simulink model "dcdc_zvs_full_bridge"  (R2026b)
settings: Solver=ode23tb  StopTime=simlength  FixedStep=tc  MaxStep=tc
values from neighbouring files (symbols this model uses):
  Idc_FS = max(Idab1_dc_nom,Idab2_dc_nom) * margin_factor    [init_model.m]
  L_core_length = 95    [magnetics_design_transformer.m]
  number_of_cells_2_sim = floor((Uout_nom-delta_load)/u_cell)    [init_model.m]    (also in run_sim_output_current_ctrl.m = floor((Uout_max-delta_load)/u_cell))
  Pnom = 175e3    (= 175000)    [init_model.m]
  tc = ts_dab/400    (= 5e-07)    [init_model.m]
  u_cell = 3.6    [init_model.m]
  Vdab2_dc_nom = ubattery2    (= 540)    [init_model.m]
  Vdc_FS = max(Vdab1_dc_nom,Vdab2_dc_nom) * margin_factor    [init_model.m]
libraries: fl_lib x32, nesl_utility x22, discrete_time_low_pass_filter x7, lithium_ion_battery x2, pi_ctrl x2, full_bridge_diode_rectifier x2, full_bridge_zvs_pwm_modulator x1, full_bridge_ideal_switch x1, full_bridge_igbt_based_with_thermal_model x1, full_bridge_mosfet_based_with_thermal_model_zvs x1, three_windings_transformer x1
(part 2 of 2)

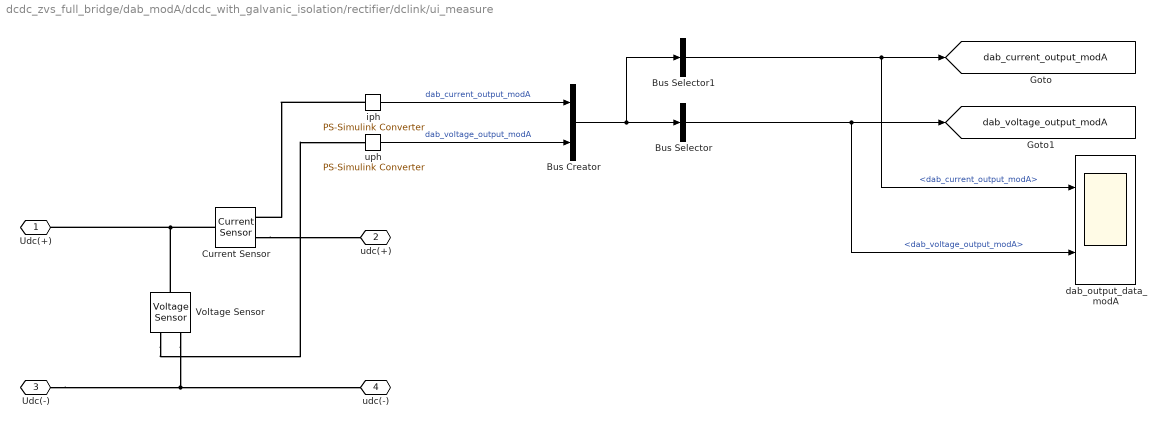
== system dcdc_zvs_full_bridge/dab_modA/dcdc_with_galvanic_isolation/rectifier/dclink/ui_measure ==
  Bus Creator : BusCreator  Inputs=2
  Bus Selector : BusSelector  OutputSignals=dab_voltage_output_modA
  Bus Selector1 : BusSelector  OutputSignals=dab_current_output_modA
  Current Sensor : fl_lib/Electrical/Electrical Sensors/Current Sensor
  Voltage Sensor : fl_lib/Electrical/Electrical Sensors/Voltage Sensor
  dab_output_data_modA : Scope  NumInputPorts=2
      settings: SampleTime=tc  ActiveDisplayYMinimum=283.61167297568261  ActiveDisplayYMaximum=358.14263055151184  DataLoggingVariableName=ScopeData11
  iph : nesl_utility/PS-Simulink Converter  PhysicalDomain=network_engine_domain  SubClassName=ps_output  LeftPortType=input  RightPortType=output  PseudoPeriodic=off  Frequencies=[]  VectorFormat=1-D array  Unit=A  AffineConversion=off
  uph : nesl_utility/PS-Simulink Converter  PhysicalDomain=network_engine_domain  SubClassName=ps_output  LeftPortType=input  RightPortType=output  PseudoPeriodic=off  Frequencies=[]  VectorFormat=1-D array  Unit=V  AffineConversion=off
  Udc(+) : PMIOPort  Side=Left
  udc(+) : PMIOPort  Port=2  Side=Right
  Udc(-) : PMIOPort  Port=3  Side=Left
  udc(-) : PMIOPort  Port=4  Side=Right
  tag scope: dab_current_output_modA=global, dab_voltage_output_modA=global
  wires:
  Bus Creator/1 -> Bus Selector1/1, Bus Selector/1
  iph/1 -> Bus Creator/1  "dab_current_output_modA"
  uph/1 -> Bus Creator/2  "dab_voltage_output_modA"
  Bus Selector1/1 -> [dab_current_output_modA], dab_output_data_modA/1  "<dab_current_output_modA>"
  Bus Selector/1 -> [dab_voltage_output_modA], dab_output_data_modA/2  "<dab_voltage_output_modA>"
  connections:
  iph/LConn1 -- Current Sensor/RConn1
  Voltage Sensor/LConn1 -- Current Sensor/LConn1 -- Udc(+)/RConn1
  Current Sensor/RConn2 -- udc(+)/RConn1
  Voltage Sensor/RConn1 -- uph/LConn1
  Voltage Sensor/RConn2 -- Udc(-)/RConn1 -- udc(-)/RConn1

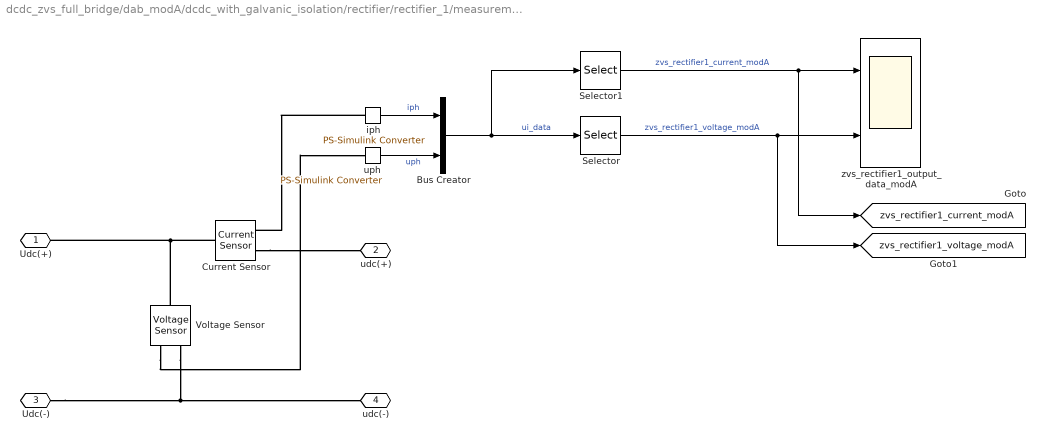
== system dcdc_zvs_full_bridge/dab_modA/dcdc_with_galvanic_isolation/rectifier/rectifier_1/measurements_rectifier_output_1 ==
  Bus Creator : BusCreator  Inputs=2
  Current Sensor : fl_lib/Electrical/Electrical Sensors/Current Sensor
  Selector : Selector  InputPortWidth=2  IndexOptions=Index vector (dialog)  Indices=2  OutputSizes=1  RuntimeRangeChecks=off
  Selector1 : Selector  InputPortWidth=2  IndexOptions=Index vector (dialog)  Indices=1  OutputSizes=1  RuntimeRangeChecks=off
  Voltage Sensor : fl_lib/Electrical/Electrical Sensors/Voltage Sensor
  iph : nesl_utility/PS-Simulink Converter  PhysicalDomain=network_engine_domain  SubClassName=ps_output  LeftPortType=input  RightPortType=output  PseudoPeriodic=off  Frequencies=[]  VectorFormat=1-D array  Unit=A  AffineConversion=off
  uph : nesl_utility/PS-Simulink Converter  PhysicalDomain=network_engine_domain  SubClassName=ps_output  LeftPortType=input  RightPortType=output  PseudoPeriodic=off  Frequencies=[]  VectorFormat=1-D array  Unit=V  AffineConversion=off
  zvs_rectifier1_output_data_modA : Scope  NumInputPorts=2
      settings: SampleTime=tc  ActiveDisplayYMinimum=-126.83833202722374  ActiveDisplayYMaximum=1141.4829766347427  DataLoggingVariableName=ScopeData2
  Udc(+) : PMIOPort  Side=Left
  udc(+) : PMIOPort  Port=2  Side=Right
  Udc(-) : PMIOPort  Port=3  Side=Left
  udc(-) : PMIOPort  Port=4  Side=Right
  tag scope: zvs_rectifier1_current_modA=global, zvs_rectifier1_voltage_modA=global
  wires:
  Bus Creator/1 -> Selector/1, Selector1/1  "ui_data"
  iph/1 -> Bus Creator/1  "iph"
  uph/1 -> Bus Creator/2  "uph"
  Selector1/1 -> [zvs_rectifier1_current_modA], zvs_rectifier1_output_data_modA/1  "zvs_rectifier1_current_modA"
  Selector/1 -> [zvs_rectifier1_voltage_modA], zvs_rectifier1_output_data_modA/2  "zvs_rectifier1_voltage_modA"
  connections:
  iph/LConn1 -- Current Sensor/RConn1
  Voltage Sensor/LConn1 -- Current Sensor/LConn1 -- Udc(+)/RConn1
  Current Sensor/RConn2 -- udc(+)/RConn1
  Voltage Sensor/RConn1 -- uph/LConn1
  Voltage Sensor/RConn2 -- Udc(-)/RConn1 -- udc(-)/RConn1

== system dcdc_zvs_full_bridge/dab_modA/dcdc_with_galvanic_isolation/rectifier/rectifier_2/measurements_rectifier_output_1 ==
  Bus Creator : BusCreator  Inputs=2
  Current Sensor : fl_lib/Electrical/Electrical Sensors/Current Sensor
  Selector : Selector  InputPortWidth=2  IndexOptions=Index vector (dialog)  Indices=2  OutputSizes=1  RuntimeRangeChecks=off
  Selector1 : Selector  InputPortWidth=2  IndexOptions=Index vector (dialog)  Indices=1  OutputSizes=1  RuntimeRangeChecks=off
  Voltage Sensor : fl_lib/Electrical/Electrical Sensors/Voltage Sensor
  iph : nesl_utility/PS-Simulink Converter  PhysicalDomain=network_engine_domain  SubClassName=ps_output  LeftPortType=input  RightPortType=output  PseudoPeriodic=off  Frequencies=[]  VectorFormat=1-D array  Unit=A  AffineConversion=off
  uph : nesl_utility/PS-Simulink Converter  PhysicalDomain=network_engine_domain  SubClassName=ps_output  LeftPortType=input  RightPortType=output  PseudoPeriodic=off  Frequencies=[]  VectorFormat=1-D array  Unit=V  AffineConversion=off
  zvs_rectifier1_output_data_modA : Scope  NumInputPorts=2
      settings: SampleTime=tc  ActiveDisplayYMinimum=-126.83833202722374  ActiveDisplayYMaximum=1141.4829766347427  DataLoggingVariableName=ScopeData2
  Udc(+) : PMIOPort  Side=Left
  udc(+) : PMIOPort  Port=2  Side=Right
  Udc(-) : PMIOPort  Port=3  Side=Left
  udc(-) : PMIOPort  Port=4  Side=Right
  tag scope: zvs_rectifier2_current_modA=global, zvs_rectifier2_voltage_modA=global
  wires:
  Selector/1 -> zvs_rectifier1_output_data_modA/2, [zvs_rectifier2_voltage_modA]  "zvs_rectifier1_voltage_modA"
  Selector1/1 -> zvs_rectifier1_output_data_modA/1, [zvs_rectifier2_current_modA]  "zvs_rectifier1_current_modA"
  uph/1 -> Bus Creator/2  "uph"
  iph/1 -> Bus Creator/1  "iph"
  Bus Creator/1 -> Selector1/1, Selector/1  "ui_data"
  connections:
  udc(-)/RConn1 -- Udc(-)/RConn1 -- Voltage Sensor/RConn2
  Voltage Sensor/RConn1 -- uph/LConn1
  Current Sensor/RConn2 -- udc(+)/RConn1
  Udc(+)/RConn1 -- Current Sensor/LConn1 -- Voltage Sensor/LConn1
  iph/LConn1 -- Current Sensor/RConn1
